simulink model "DI_triger"  (R2023a)
settings: Solver=ode4  StartTime=0.0  StopTime=inf  FixedStep=0.01  RelTol=1e-3
libraries: ASEToolBox x3, etargetslib x2, simulink x1
settings Model: Creator=admin  LastModifiedBy=LENOVO
settings DataIOCC: SaveOutput=off  SignalLogging=off  SaveTime=off
settings OptimizationCC: EnhancedBackFolding=on  PassReuseOutputArgsAs=Individual arguments  ZeroExternalMemoryAtStartup=off  ZeroInternalMemoryAtStartup=off  OptimizeBlockOrder=speed  DifferentSizesBufferReuse=on  OptimizationCustomize=off  EfficientTunableParamExpr=on
settings DebuggingCC: ParameterTunabilityLossMsg=error
settings HardwareCC: ProdBitPerLong=64  ProdHWDeviceType=Intel->x86-64 (Linux 64)
settings SFSimCC: MATLABDynamicMemAlloc=off
settings RTWCC: Description=Embedded Coder  SystemTargetFile=ert.tlc  GenCodeOnly=on  TemplateMakefile=ert_default_tmf  RetainRTWFile=on
settings CodeAppCC: ForceParamTrailComments=on  IgnoreCustomStorageClasses=off  OperatorAnnotations=on  SimulinkDataObjDesc=on  SFDataObjDesc=on  InsertBlockDesc=on
settings ERTTargetCC: TargetLangStandard=C99 (ISO)  SupportContinuousTime=on  RTWCAPISignals=on  RTWCAPIParams=on  RTWCAPIStates=on  RTWCAPIRootIO=on  ERTCustomFileTemplate=example_file_process.tlc

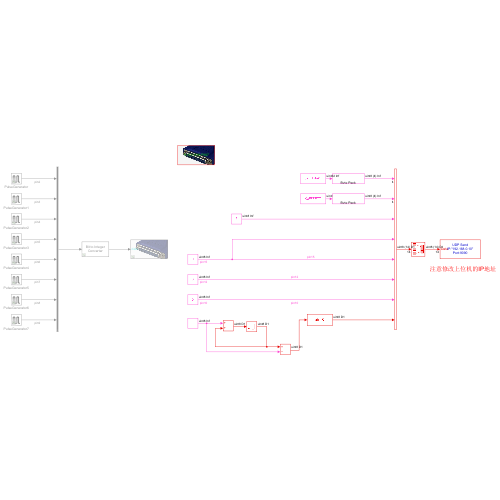
[thumbnail: Simulink's stored preview of the top-level diagram]
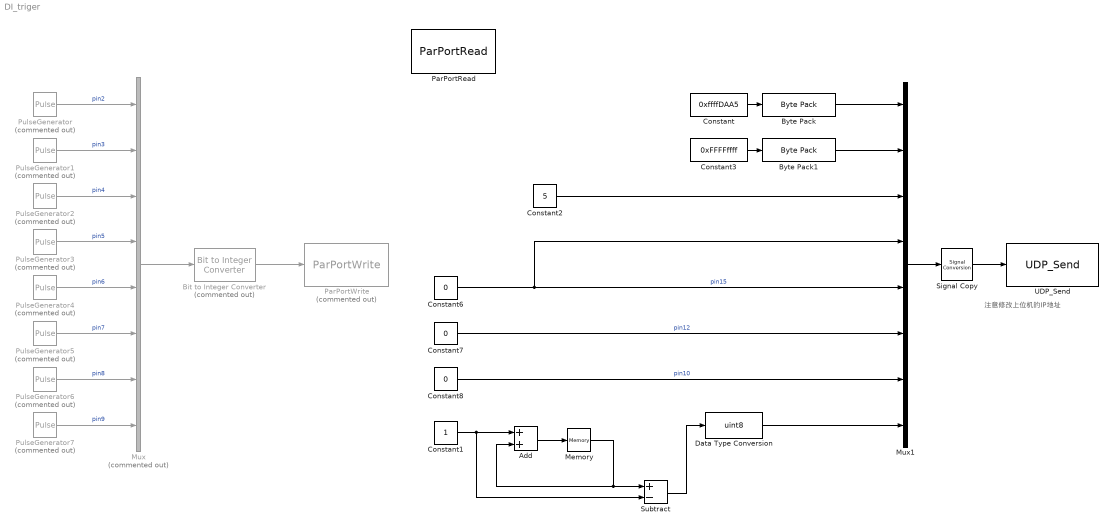
== system DI_triger ==
  note: 注意修改上位机的IP地址
  Add : Sum
  Bit to Integer Converter : simulink/Logic and Bit Operations/Bit to Integer Converter  Commented=on  nbits=8  bitOrder=LSB first  signedOutputValues=Unsigned  outDtype=uint8  outDtypeSigned=Inherit via internal rule
  Byte Pack : etargetslib/Byte Pack  datatypes={'uint32'}  byteAlign=1
  Byte Pack1 : etargetslib/Byte Pack  datatypes={'uint32'}  byteAlign=1
  Constant : Constant  Value=0xffffDAA5  OutDataTypeStr=uint32
  Constant1 : Constant  OutDataTypeStr=uint8
  Constant2 : Constant  Value=5  OutDataTypeStr=uint8
  Constant3 : Constant  Value=0xFFFFffff  OutDataTypeStr=uint32
  Constant6 : Constant  Value=0  OutDataTypeStr=uint8
  Constant7 : Constant  Value=0  OutDataTypeStr=uint8
  Constant8 : Constant  Value=0  OutDataTypeStr=uint8
  Data Type Conversion : DataTypeConversion  OutDataTypeStr=uint8  SaturateOnIntegerOverflow=off  RndMeth=Floor
  Memory : Memory
  Mux : Mux  Commented=on  Inputs=8
  Mux1 : Mux  Inputs=8
  ParPortRead : ASEToolBox/DIOModule/ParPortRead  g_par_select=/dev/parport0  g_ext_trigger=on  g_pin=PIN7
      settings: SourceProductName=ASEToolBox
  ParPortWrite : ASEToolBox/DIOModule/ParPortWrite  Commented=on  g_par_select=/dev/parport0
      settings: SourceProductName=ASEToolBox
  PulseGenerator : DiscretePulseGenerator  Commented=on  PulseType=Time based  Period=0.04  PulseWidth=25
  PulseGenerator1 : DiscretePulseGenerator  Commented=on  PulseType=Time based  Period=0.1  PulseWidth=20
  PulseGenerator2 : DiscretePulseGenerator  Commented=on  PulseType=Time based  Period=0.1  PulseWidth=30
  PulseGenerator3 : DiscretePulseGenerator  Commented=on  PulseType=Time based  Period=0.1  PulseWidth=40
  PulseGenerator4 : DiscretePulseGenerator  Commented=on  PulseType=Time based  Period=0.1  PulseWidth=50
  PulseGenerator5 : DiscretePulseGenerator  Commented=on  PulseType=Time based  Period=0.1  PulseWidth=60
  PulseGenerator6 : DiscretePulseGenerator  Commented=on  PulseType=Time based  Period=0.1  PulseWidth=70
  PulseGenerator7 : DiscretePulseGenerator  Commented=on  PulseType=Time based  Period=0.1  PulseWidth=80
  Signal Copy : SignalConversion  OverrideOpt=on
  Subtract : Sum  Inputs=+-
  UDP_Send : ASEToolBox/UDPModule/UDP_Send  Priority=0  g_localIP="\"192.168.0.7\""  g_localPort=8080  g_ip="\"192.168.0.10\""  g_port=9090  g_buffersize=14
      settings: SourceProductName=ASEToolBox
  wires:
  PulseGenerator/1 -> Mux/1  "pin2"
  PulseGenerator1/1 -> Mux/2  "pin3"
  PulseGenerator2/1 -> Mux/3  "pin4"
  PulseGenerator3/1 -> Mux/4  "pin5"
  PulseGenerator7/1 -> Mux/8  "pin9"
  PulseGenerator6/1 -> Mux/7  "pin8"
  PulseGenerator5/1 -> Mux/6  "pin7"
  PulseGenerator4/1 -> Mux/5  "pin6"
  Bit to Integer Converter/1 -> ParPortWrite/1
  Mux/1 -> Bit to Integer Converter/1
  Constant8/1 -> Mux1/7  "pin10"
  Mux1/1 -> Signal Copy/1
  Byte Pack/1 -> Mux1/1
  Constant/1 -> Byte Pack/1
  Signal Copy/1 -> UDP_Send/1
  Constant6/1 -> Mux1/4, Mux1/5  "pin15"
  Constant7/1 -> Mux1/6  "pin12"
  Constant3/1 -> Byte Pack1/1
  Byte Pack1/1 -> Mux1/2
  Constant2/1 -> Mux1/3
  Constant1/1 -> Subtract/2, Add/1
  Data Type Conversion/1 -> Mux1/8
  Memory/1 -> Subtract/1, Add/2
  Add/1 -> Memory/1
  Subtract/1 -> Data Type Conversion/1
